simulink model "G11_Simulink"  (R2026a)
settings: Solver=ode4  StopTime=900  FixedStep=0.005
libraries: cstblocks_lti x1
settings Model: Creator=nelis  LastModifiedBy=nelis

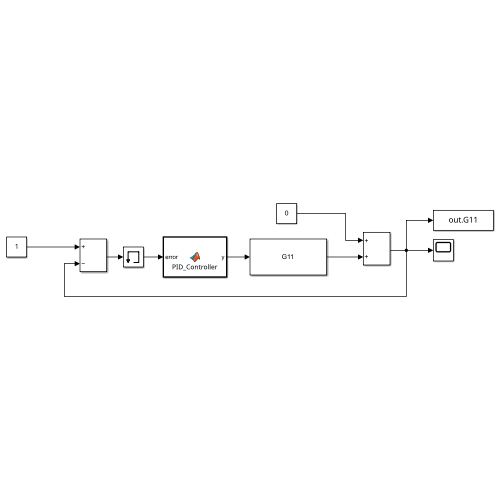
[thumbnail: Simulink's stored preview of the top-level diagram]
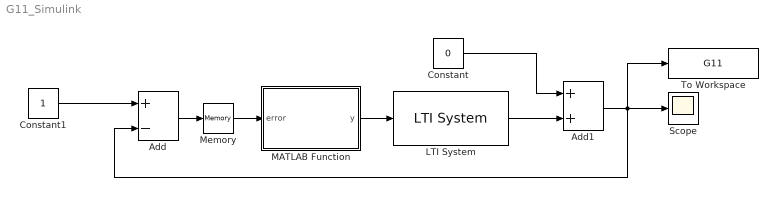
== system G11_Simulink ==
  Add : Sum  Inputs=+-
  Add1 : Sum
  Constant : Constant  Value=0
  Constant1 : Constant
  LTI System : cstblocks_lti/LTI System  sys=G11  IC=[]  PadeOrder=1
      settings: LibrarySourceBlock=cstblocks/LTI System
  MATLAB Function : MATLAB Function  TreatAsAtomicUnit=on  SystemSampleTime=0.005
  Memory : Memory
  Scope : Scope
      settings: ActiveDisplayYMinimum=-2.0998491864331172  ActiveDisplayYMaximum=2.4165756816298241
  To Workspace : ToWorkspace  VariableName=G11  SaveFormat=Timeseries  SampleTime=-1
  wires:
  MATLAB Function/1(y) -> LTI System/1
  LTI System/1 -> Add1/2
  Constant/1 -> Add1/1
  Constant1/1 -> Add/1
  Add1/1 -> To Workspace/1, Scope/1, Add/2
  Add/1 -> Memory/1
  Memory/1 -> MATLAB Function/1(error)

== matlab function G11_Simulink/MATLAB Function ==
  data: y output; error input
function y =  PID_Controller(error)
    persistent prev_error;
    persistent integral;
    dt = 0.005;

    D = 1.1792;
    P = 0.1295055;
    I = 0.00295055;

    if isempty(prev_error)
        prev_error = error;
    end

    if isempty(integral)
        integral = 0;
    end

    next_integral = integral + error * dt;
    derivative = (error - prev_error)/dt;

    pid_out = P*error + I*next_integral + D*derivative;

    if pid_out >= 3.3
        pid_out = 3.3;
        if error < 0
            integral = next_integral;
        end

    elseif pid_out < 0
        pid_out = 0;
        if error > 0
            integral = next_integral;
        end
    else
        integral = next_integral;
    end

    prev_error = error;

y = pid_out;
